simulink model "hopper_6dof_NED_fault_injection"  (R2026a)
settings: Solver=FixedStepAuto  StopTime=30  FixedStep=1e-3  RelTol=1e-5
values from neighbouring files (symbols this model uses):
  cg_init = MP.cg_init    [cg_moi_test.m]
  dcg_dMfu_table = [-0.00217262899893 -0.00217440598527 -0.00217621044518 -0.00217804213665 -0.0021799008032 -0.00218178621725 -0.00218369812677 -0.0021856362975 -0.00218760049076 -0.00218959047338 -0.00219160600889 -0.0021936468686 ... (10000 elements, 100x100)]    [cg_I_LUT.mat]    (also in cg_moi_table_generation.m = MP.dcg_dMfu_table; cg_moi_test.m = MP.dcg_dMfu_table)
  dcg_dMox_table = [0.00344752331682 0.00347104712195 0.00349447366155 0.00351780347518 0.00354103709244 0.00356417504177 0.00358721784832 0.00361016603279 0.00363302011142 0.00365578059713 0.00367844800397 0.0037010228382 ... (10000 elements, 100x100)]    [cg_I_LUT.mat]    (also in cg_moi_table_generation.m = MP.dcg_dMox_table; cg_moi_test.m = MP.dcg_dMox_table)
  dI_dMfu_table = [0.00582660125037 0.00582660125148 0.00582660125148 0.00582660125037 0.00582660125037 0.00582660124926 0.00582660124926 0.00582660125037 0.00582660125037 0.00582660125148 0.00582660125148 0.00582660125037 ... (90000 elements, 100x100x9)]    [cg_I_LUT.mat]    (also in cg_moi_table_generation.m = MP.dI_dMfu_table; cg_moi_test.m = MP.dI_dMfu_table)
  dI_dMox_table = [0.00582660125037 0.00582660124926 0.00582660125037 0.00582660124926 0.00582660125037 0.00582660124926 0.00582660125037 0.00582660124926 0.00582660125037 0.00582660125037 0.00582660125037 0.00582660125037 ... (90000 elements, 100x100x9)]    [cg_I_LUT.mat]    (also in cg_moi_table_generation.m = MP.dI_dMox_table; cg_moi_test.m = MP.dI_dMox_table)
  engine_cg = IN.engine_cg    [cg_moi_test.m]
  engine_mass = IN.engine_mass    [cg_moi_test.m]
  fu_masses = [0 0.131313131313 0.262626262626 0.393939393939 0.525252525253 0.656565656566 0.787878787879 0.919191919192 1.05050505051 1.18181818182 1.31313131313 1.44444444444 ... (100 elements, 1x100)]    [cg_I_LUT.mat]    (also in cg_moi_table_generation.m = MP.fu_masses; cg_moi_test.m = MP.fu_masses)
  g = p.g    [HopperLinearization_6DOF.m]    (also in HopperLinearization_6DOF_LQR.m; HopperLinearization_6DOF_inertial.m; HopperLinearization_errorq.m; TetherTrajectory.m = 9.81)
  K1flat = zeros(N,52)    [GenerateLQ.m]    (also in LQTrack_Master.m = zeros(length(tgrid),48); LinerizationMaster.m = zeros(length(tgrid),52))
  K2grid = GainTable.K2'    [GenerateLQ.m]    (also in LQTrack_Master.m; LinerizationMaster.m)
  MoI_init = MP.MoI_init    [cg_moi_test.m]
  mount_cg = IN.mount_cg    [cg_moi_test.m]
  ox_masses = [0 0.161616161616 0.323232323232 0.484848484848 0.646464646465 0.808080808081 0.969696969697 1.13131313131 1.29292929293 1.45454545455 1.61616161616 1.77777777778 ... (100 elements, 1x100)]    [cg_I_LUT.mat]    (also in cg_moi_table_generation.m = MP.ox_masses; cg_moi_test.m = MP.ox_masses)
  tank_r = 0.10795    [baffle_lut.mat]    (also in cg_moi_test.m = TANKS.singular.radius)
  Target_Trajectory = [0 0 0 0 0 0 0 0 0 sqrt(2)/2 0 sqrt(2)/2 0]'    [LQGeneral.m]    (also in LQTrack_Master.m = [x_trajectory; y_trajectory; z_trajectory;                  ; LinerizationMaster.m = [x_trajectory;y_trajectory;z_trajectory;    vx_trajectory;vy)
  tgrid = t    [LQTrack_Master.m]    (also in LinerizationMaster.m; Trajectory3.m = [t1 t2 t3]'; TrajectoryFollowingGains.m = tgrid(:); TrajectoryFollowingGains2.m = tgrid(:))
  unom = [T_profile, delta_y_profile, delta_z_profile, rcsp]    [LQTrack_Master.m]    (also in LinerizationMaster.m; Trajectory3.m = [; TrajectoryFollowingGains.m = [T_profile(:), zeros(N,1)])
undefined symbols (not defined in the file or in its folder): ENGINE, fu_axial_damping_ratios, fu_lateral_damping_ratios, fu_mass_profile, fu_mdot_data, IN, OUT, ox_axial_damping_ratios, ox_lateral_damping_ratios, ox_mass_profile, ox_mdot_data, pressureLevels, r_leg_1, r_leg_2, r_leg_3, r_leg_4, TANKS, thrust_data, uwndTable, VEH, vwndTable
libraries: fl_lib x31, nesl_utility x25, matrix_library x18, SimscapeFluids_lib x10, simulink_extras x7, slpidlib x7, simulink x7, dspindex x3, aerolibanim x1, commrandsrc3 x1, aerolibutil x1, dspsrcs4 x1
(part 6 of 7)

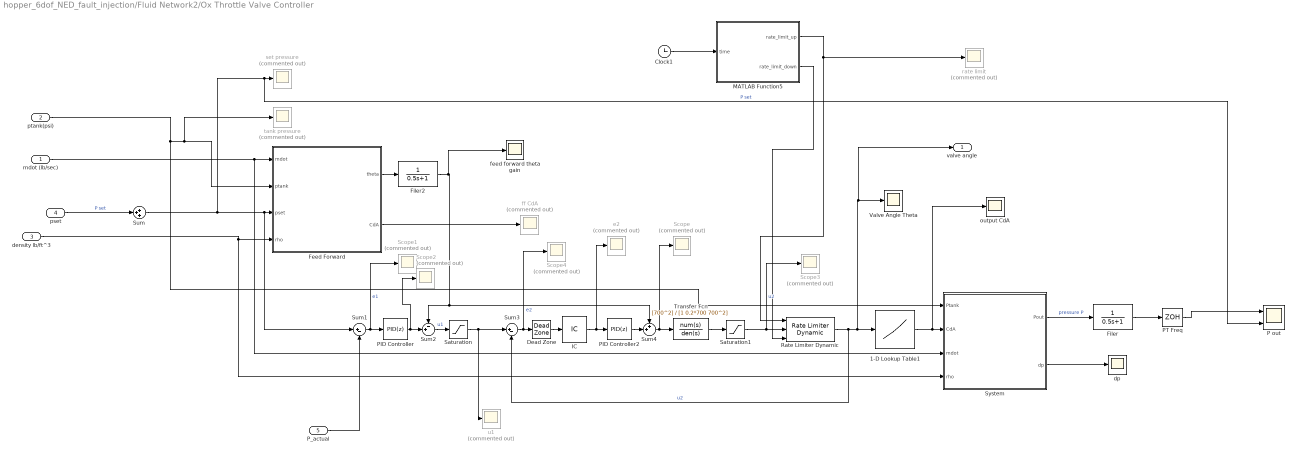
== system hopper_6dof_NED_fault_injection/Fluid Network2/Ox Throttle Valve Controller ==
  mdot (lb/sec) : Inport
  ptank(psi) : Inport  Port=2
  density lb/ft^3 : Inport  Port=3
  pset : Inport  Port=4
  P_actual : Inport  Port=5
  1-D Lookup Table1 : Lookup_n-D  NumberOfTableDimensions=1  BreakpointsForDimension1=[27, 36, 45, 54, 63, 72, 81, 90]  Table="[0.01,  0.06, 0.21, 0.46, 0.83, 1.35, 2.04, 2.93] ./ 37.97"  ExtrapMethod=Clip  InternalRulePriority=Speed  RndMeth=Simplest
  Clock1 : Clock
  Dead Zone : DeadZone  LowerValue=-30  UpperValue=30
  Feed Forward : MATLAB Function  TreatAsAtomicUnit=on
  Filer : TransferFcn  Denominator=[0.5 1]
  Filer2 : TransferFcn  Denominator=[0.5 1]
  IC : InitialCondition  Value=0
  MATLAB Function5 : MATLAB Function  TreatAsAtomicUnit=on
  P out : Scope  NumInputPorts=2
      settings: ActiveDisplayYMinimum=-153.57845403205533  ActiveDisplayYMaximum=515.02423080214487  DataLoggingVariableName=ScopeData20
  PID Controller : slpidlib/PID Controller  Controller=PID  Form=Parallel  TimeDomain=Discrete-time  UseExternalTs=off  SampleTime=0.01  IntegratorMethod=Forward Euler  FilterMethod=Forward Euler  ControllerParametersSource=internal  P=6  I=0.5  UseKiTs=off  D=0  UseExternalDerivativeSource=off  N=100  UseFilter=on  TunerSelectOption=Transfer Function Based (PID Tuner App)  InitialConditionSource=internal  InitialConditionForIntegrator=0  InitialConditionForFilter=0  DifferentiatorICPrevScaledInput=0  ExternalReset=none  TrackingMode=off  Kt=1  LimitOutput=off  SatLimitsSource=internal  UpperSaturationLimit=inf  LowerSaturationLimit=-inf  LinearizeAsGain=on  AntiWindupMode=none  Kb=1  LimitIntegrator=off  UpperIntegratorSaturationLimit=inf  LowerIntegratorSaturationLimit=-inf  POutMin=[]  POutMax=[]  IOutMin=[]  IOutMax=[]  DOutMin=[]  DOutMax=[]  NOutMin=[]  NOutMax=[]  SumOutMin=[]  SumOutMax=[]  SaturationOutMin=[]  SaturationOutMax=[]  PParamMin=[]  PParamMax=[]  IParamMin=[]  IParamMax=[]  DParamMin=[]  DParamMax=[]  NParamMin=[]  NParamMax=[]  KbParamMin=[]  KbParamMax=[]  KtParamMin=[]  KtParamMax=[]  KbOutMin=[]  KbOutMax=[]  KtOutMin=[]  KtOutMax=[]  IntegratorOutMin=[]  IntegratorOutMax=[]  FilterOutMin=[]  FilterOutMax=[]  SumI1OutMin=[]  SumI1OutMax=[]  SumI2OutMin=[]  SumI2OutMax=[]  SumI3OutMin=[]  SumI3OutMax=[]  SumI4OutMin=[]  SumI4OutMax=[]  SumDOutMin=[]  SumDOutMax=[]  DifferentiatorOutMin=[]  DifferentiatorOutMax=[]  FilterDiffOutCoefMin=[]  FilterDiffOutCoefMax=[]  ReciprocalOutMin=[]  ReciprocalOutMax=[]  SumDenOutMin=[]  SumDenOutMax=[]  SumNumOutMin=[]  SumNumOutMax=[]  DivideOutMin=[]  DivideOutMax=[]  UdiffTsProdOutMin=[]  UdiffTsProdOutMax=[]  NTsProdOutMin=[]  NTsProdOutMax=[]  UintegralTsProdOutMin=[]  UintegralTsProdOutMax=[]  UngainTsProdOutMin=[]  UngainTsProdOutMax=[]  ClampingZeroOutDataTypeStr=Inherit: Inherit via back propagation  ClampingZeroOutMin=[]  ClampingZeroOutMax=[]  FilterDenConstantOutDataTypeStr=Inherit: Inherit via back propagation  FilterDenConstantOutMin=[]  FilterDenConstantOutMax=[]  PCopyOutDataTypeStr=Inherit: Inherit via back propagation  PCopyOutMin=[]  PCopyOutMax=[]  NCopyOutDataTypeStr=Inherit: Inherit via back propagation  NCopyOutMin=[]  NCopyOutMax=[]  IntegratorContinuousStateAttributes=''  IntegratorStateMustResolveToSignalObject=off  IntegratorRTWStateStorageClass=Auto  FilterContinuousStateAttributes=''  FilterStateMustResolveToSignalObject=off  FilterRTWStateStorageClass=Auto  ParallelPVariant=InternalParameters  IdealPVariant=Disabled  IVariant=InternalParameters  DVariant=InternalParameters  IntegratorVariant=Discrete  SatVariant=Disabled  AWVariant=Passthrough  PCopyVariant=Disabled  TRVariant=Disabled  FdbkBlocksVariant=Forward  IdealPFdbkVariant=Disabled  SatFdbkVariant=Disabled  DerivativeFilterVariant=ForwardEulerFilter  NVariant=InternalParameters  NCopyVariant=Disabled  FilterICVariant=InternalICsFilter  IntegratorICVariant=InternalICs  ExternalResetVariant=Disabled  TRSumVariant=Passthrough  SumFdbkVariant=Disabled  SumVariant=Sum_PID  TsampFilterVariant=InternalTs  TsampNgainVariant=Passthrough  TsampIntegralVariant=Disabled_SignalSpec  ExternalSaturationOutDataTypeStr=Inherit: Same as second input  DerivativeSourceVariant=ErrorSignal  PreIntVariant=InternalPreInt
  PID Controller2 : slpidlib/PID Controller  Controller=PID  Form=Parallel  TimeDomain=Discrete-time  UseExternalTs=off  SampleTime=0.001  IntegratorMethod=Forward Euler  FilterMethod=Forward Euler  ControllerParametersSource=internal  P=0.1  I=0.6  UseKiTs=off  D=0  UseExternalDerivativeSource=off  N=100  UseFilter=on  TunerSelectOption=Transfer Function Based (PID Tuner App)  InitialConditionSource=internal  InitialConditionForIntegrator=0  InitialConditionForFilter=0  DifferentiatorICPrevScaledInput=0  ExternalReset=none  TrackingMode=off  Kt=1  LimitOutput=off  SatLimitsSource=internal  UpperSaturationLimit=inf  LowerSaturationLimit=-inf  LinearizeAsGain=on  AntiWindupMode=none  Kb=1  LimitIntegrator=off  UpperIntegratorSaturationLimit=inf  LowerIntegratorSaturationLimit=-inf  POutMin=[]  POutMax=[]  IOutMin=[]  IOutMax=[]  DOutMin=[]  DOutMax=[]  NOutMin=[]  NOutMax=[]  SumOutMin=[]  SumOutMax=[]  SaturationOutMin=[]  SaturationOutMax=[]  PParamMin=[]  PParamMax=[]  IParamMin=[]  IParamMax=[]  DParamMin=[]  DParamMax=[]  NParamMin=[]  NParamMax=[]  KbParamMin=[]  KbParamMax=[]  KtParamMin=[]  KtParamMax=[]  KbOutMin=[]  KbOutMax=[]  KtOutMin=[]  KtOutMax=[]  IntegratorOutMin=[]  IntegratorOutMax=[]  FilterOutMin=[]  FilterOutMax=[]  SumI1OutMin=[]  SumI1OutMax=[]  SumI2OutMin=[]  SumI2OutMax=[]  SumI3OutMin=[]  SumI3OutMax=[]  SumI4OutMin=[]  SumI4OutMax=[]  SumDOutMin=[]  SumDOutMax=[]  DifferentiatorOutMin=[]  DifferentiatorOutMax=[]  FilterDiffOutCoefMin=[]  FilterDiffOutCoefMax=[]  ReciprocalOutMin=[]  ReciprocalOutMax=[]  SumDenOutMin=[]  SumDenOutMax=[]  SumNumOutMin=[]  SumNumOutMax=[]  DivideOutMin=[]  DivideOutMax=[]  UdiffTsProdOutMin=[]  UdiffTsProdOutMax=[]  NTsProdOutMin=[]  NTsProdOutMax=[]  UintegralTsProdOutMin=[]  UintegralTsProdOutMax=[]  UngainTsProdOutMin=[]  UngainTsProdOutMax=[]  ClampingZeroOutDataTypeStr=Inherit: Inherit via back propagation  ClampingZeroOutMin=[]  ClampingZeroOutMax=[]  FilterDenConstantOutDataTypeStr=Inherit: Inherit via back propagation  FilterDenConstantOutMin=[]  FilterDenConstantOutMax=[]  PCopyOutDataTypeStr=Inherit: Inherit via back propagation  PCopyOutMin=[]  PCopyOutMax=[]  NCopyOutDataTypeStr=Inherit: Inherit via back propagation  NCopyOutMin=[]  NCopyOutMax=[]  IntegratorContinuousStateAttributes=''  IntegratorStateMustResolveToSignalObject=off  IntegratorRTWStateStorageClass=Auto  FilterContinuousStateAttributes=''  FilterStateMustResolveToSignalObject=off  FilterRTWStateStorageClass=Auto  ParallelPVariant=InternalParameters  IdealPVariant=Disabled  IVariant=InternalParameters  DVariant=InternalParameters  IntegratorVariant=Discrete  SatVariant=Disabled  AWVariant=Passthrough  PCopyVariant=Disabled  TRVariant=Disabled  FdbkBlocksVariant=Forward  IdealPFdbkVariant=Disabled  SatFdbkVariant=Disabled  DerivativeFilterVariant=ForwardEulerFilter  NVariant=InternalParameters  NCopyVariant=Disabled  FilterICVariant=InternalICsFilter  IntegratorICVariant=InternalICs  ExternalResetVariant=Disabled  TRSumVariant=Passthrough  SumFdbkVariant=Disabled  SumVariant=Sum_PID  TsampFilterVariant=InternalTs  TsampNgainVariant=Passthrough  TsampIntegralVariant=Disabled_SignalSpec  ExternalSaturationOutDataTypeStr=Inherit: Same as second input  DerivativeSourceVariant=ErrorSignal  PreIntVariant=InternalPreInt
  PT Freq : ZeroOrderHold  SampleTime=1/200
  Rate Limiter Dynamic : simulink/Discontinuities/Rate Limiter Dynamic
  Saturation : Saturate  UpperLimit=90  LowerLimit=0
  Saturation1 : Saturate  UpperLimit=90  LowerLimit=0
  Scope{,1..4} (5 alike) : Scope  Commented=on
      Scope settings: ActiveDisplayYMinimum=-275.11641924282065  ActiveDisplayYMaximum=563.35245614782866  DataLoggingVariableName=ScopeData23
      Scope1 settings: ActiveDisplayYMinimum=-63.640747784829  ActiveDisplayYMaximum=395.9600830872032  DataLoggingVariableName=ScopeData24
      Scope2 settings: ActiveDisplayYMinimum=-1  ActiveDisplayYMaximum=1  DataLoggingVariableName=ScopeData25
      Scope3 settings: ActiveDisplayYMinimum=-1  ActiveDisplayYMaximum=1  DataLoggingVariableName=ScopeData26
      Scope4 settings: ActiveDisplayYMinimum=-1  ActiveDisplayYMaximum=1  DataLoggingVariableName=ScopeData27
  Sum : Sum  Inputs=+++
  Sum1 : Sum  Inputs=|+-
  Sum2 : Sum  Inputs=-+|
  Sum3 : Sum  Inputs=|+-
  Sum4 : Sum  Inputs=++|
  System : MATLAB Function  TreatAsAtomicUnit=on
  Transfer Fcn : TransferFcn  Numerator=[700^2]  Denominator=[1 0.2*700 700^2]
  Valve Angle Theta : Scope
      settings: ActiveDisplayYMinimum=-54.50975234839  ActiveDisplayYMaximum=77.0496336171224
  dp : Scope
      settings: ActiveDisplayYMinimum=-18119.240749435841  ActiveDisplayYMaximum=163753.70976632342  DataLoggingVariableName=ScopeData28
  e2 : Scope  Commented=on
      settings: ActiveDisplayYMinimum=-94.713391249832966  ActiveDisplayYMaximum=253.61308310962266  DataLoggingVariableName=ScopeData29
  feed forward theta gain : Scope
      settings: ActiveDisplayYMinimum=36.144112332478429  ActiveDisplayYMaximum=40.8018145520034  DataLoggingVariableName=ScopeData2
  ff CdA : Scope  Commented=on
      settings: ActiveDisplayYMinimum=0.00619  ActiveDisplayYMaximum=0.00757  DataLoggingVariableName=ScopeData30
  output CdA : Scope
      settings: ActiveDisplayYMinimum=-0.0014226243070618195  ActiveDisplayYMaximum=0.015437276914728357  DataLoggingVariableName=ScopeData3
  rate limit : Scope  Commented=on
      settings: ActiveDisplayYMinimum=-1  ActiveDisplayYMaximum=1  DataLoggingVariableName=ScopeData31
  set pressure : Scope  Commented=on
      settings: ActiveDisplayYMinimum=-1  ActiveDisplayYMaximum=1  DataLoggingVariableName=ScopeData32
  tank pressure : Scope  Commented=on
      settings: ActiveDisplayYMinimum=243.75  ActiveDisplayYMaximum=306.25  DataLoggingVariableName=ScopeData33
  u1 : Scope  Commented=on
      settings: ActiveDisplayYMinimum=-1  ActiveDisplayYMaximum=1  DataLoggingVariableName=ScopeData34
  valve angle : Outport
  wires:
  Sum3/1 -> Dead Zone/1, Scope4/1  "e2"
  density lb/ft^3/1 -> System/4(rho), Feed Forward/4(rho)
  Filer/1 -> PT Freq/1
  Sum/1 -> P out/2, set pressure/1, Sum1/1, Feed Forward/3(pset)  "P set"
  ptank(psi)/1 -> System/1(Ptank), Feed Forward/2(ptank), tank pressure/1
  PID Controller/1 -> Scope2/1, Sum2/2
  PT Freq/1 -> P out/1
  Transfer Fcn/1 -> Saturation1/1
  IC/1 -> PID Controller2/1, e2/1
  Feed Forward/1(theta) -> Filer2/1
  MATLAB Function5/2(rate_limit_down) -> Rate Limiter Dynamic/3
  Dead Zone/1 -> IC/1
  Rate Limiter Dynamic/1 -> valve angle/1, Valve Angle Theta/1, 1-D Lookup Table1/1, Sum3/2  "u2"
  pset/1 -> Sum/2  "P set"
  Sum4/1 -> Scope/1, Transfer Fcn/1
  Saturation1/1 -> Scope3/1, Rate Limiter Dynamic/2  "u2"
  mdot (lb/sec)/1 -> System/3(mdot), Feed Forward/1(mdot)
  MATLAB Function5/1(rate_limit_up) -> Rate Limiter Dynamic/1, rate limit/1
  Clock1/1 -> MATLAB Function5/1(time)
  1-D Lookup Table1/1 -> System/2(CdA), output CdA/1
  PID Controller2/1 -> Sum4/2
  Sum1/1 -> Scope1/1, PID Controller/1  "e1"
  Sum2/1 -> Saturation/1  "u1"
  Feed Forward/2(CdA) -> ff CdA/1
  System/2(dp) -> dp/1
  Saturation/1 -> u1/1, Sum3/1
  System/1(Pout) -> Filer/1  "pressure P"
  Filer2/1 -> Sum4/1, Sum2/1, feed forward theta gain/1
  P_actual/1 -> Sum1/2

== system hopper_6dof_NED_fault_injection/Fluid Network2/Physical Combustion Chamber ==
  pc : Inport
  Local Restriction (TL) : fl_lib/Thermal Liquid/Elements/Local Restriction (TL)  Commented=through  restriction_type=foundation.enum.restriction_type.fixed  restriction_area=0.001 m^2  min_area=1e-10 m^2  max_area=0.005 m^2  area=0.01 m^2  Cd=0.64  Re_c=150  pressure_recovery=true
  Local Restriction (TL)1 : fl_lib/Thermal Liquid/Elements/Local Restriction (TL)  Commented=through  restriction_type=foundation.enum.restriction_type.fixed  restriction_area=0.001 m^2  min_area=1e-10 m^2  max_area=0.005 m^2  area=0.01 m^2  Cd=0.64  Re_c=150  pressure_recovery=true
  Pressure Source (TL) : fl_lib/Thermal Liquid/Sources/Pressure Source (TL)  source_type=foundation.enum.constant_controlled.controlled  pressure_differential=0 MPa  power_spec=foundation.enum.power_spec.isentropic  area=0.01 m^2
      settings: InternalSimscapePortConfiguration="{\"Bottom\":[],\"Left\":[{\"id\":\"A\",\"label\":\"A\",\"type\":\"foundation.thermal_liquid.thermal_liquid\"},{\"id\":\"P\",\"label\":\"P\",\"type\":\"input\"}],\"Right\":[{\"id\":\"B\",\"label\":\"B\",\"type\":\"foundation.thermal_liquid.thermal_liquid\"}],\"Top\":[]}"
  Pressure Source (TL)1 : fl_lib/Thermal Liquid/Sources/Pressure Source (TL)  source_type=foundation.enum.constant_controlled.controlled  pressure_differential=0 MPa  power_spec=foundation.enum.power_spec.isentropic  area=0.01 m^2
      settings: InternalSimscapePortConfiguration="{\"Bottom\":[],\"Left\":[{\"id\":\"A\",\"label\":\"A\",\"type\":\"foundation.thermal_liquid.thermal_liquid\"},{\"id\":\"P\",\"label\":\"P\",\"type\":\"input\"}],\"Right\":[{\"id\":\"B\",\"label\":\"B\",\"type\":\"foundation.thermal_liquid.thermal_liquid\"}],\"Top\":[]}"
  Reservoir (TL) : fl_lib/Thermal Liquid/Elements/Reservoir (TL)  pressure_spec=foundation.enum.pressure_spec.atmospheric  reservoir_pressure=0.101325 MPa  reservoir_temperature=293.15 K  area=0.01 m^2
  Reservoir (TL)1 : fl_lib/Thermal Liquid/Elements/Reservoir (TL)  pressure_spec=foundation.enum.pressure_spec.atmospheric  reservoir_pressure=0.101325 MPa  reservoir_temperature=100 K  area=0.01 m^2
  Simulink-PS Converter1 : nesl_utility/Simulink-PS Converter  PhysicalDomain=network_engine_domain  SubClassName=ps_input  LeftPortType=input  RightPortType=output  PseudoPeriodic=off  Frequencies=[]  NoiseDistribution=none  NoiseParameters=[]  Unit=1  AffineConversion=off  FilteringAndDerivatives=filter  SimscapeFilterOrder=1  InputFilterTimeConstant=0.001  UdotUserProvided=0
  Simulink-PS Converter4 : nesl_utility/Simulink-PS Converter  PhysicalDomain=network_engine_domain  SubClassName=ps_input  LeftPortType=input  RightPortType=output  PseudoPeriodic=off  Frequencies=[]  NoiseDistribution=none  NoiseParameters=[]  Unit=1  AffineConversion=off  FilteringAndDerivatives=filter  SimscapeFilterOrder=1  InputFilterTimeConstant=0.001  UdotUserProvided=0
  fuel line : PMIOPort  Side=Right
  ox line : PMIOPort  Port=2  Side=Right
  wires:
  pc/1 -> Simulink-PS Converter1/1, Simulink-PS Converter4/1
  connections:
  Simulink-PS Converter4/RConn1 -- Pressure Source (TL)/LConn2
  Simulink-PS Converter1/RConn1 -- Pressure Source (TL)1/LConn2
  Local Restriction (TL)/LConn1 -- Pressure Source (TL)/LConn1
  Reservoir (TL)/LConn1 -- Local Restriction (TL)/RConn1
  fuel line/RConn1 -- Pressure Source (TL)/RConn1
  Local Restriction (TL)1/LConn1 -- Pressure Source (TL)1/LConn1
  Reservoir (TL)1/LConn1 -- Local Restriction (TL)1/RConn1
  Pressure Source (TL)1/RConn1 -- ox line/RConn1

== system hopper_6dof_NED_fault_injection/Fluid Network2/fuel mdot feedback//corrections ==
  actual mdot : Inport
  commanded mdot : Inport  Port=2
  MR correction : Inport  Port=3
  PID Controller1 : slpidlib/PID Controller  Controller=PID  Form=Parallel  TimeDomain=Continuous-time  UseExternalTs=off  SampleTime=-1  IntegratorMethod=Forward Euler  FilterMethod=Forward Euler  ControllerParametersSource=internal  P=1  I=1  UseKiTs=off  D=0  UseExternalDerivativeSource=off  N=20  UseFilter=on  TunerSelectOption=Transfer Function Based (PID Tuner App)  InitialConditionSource=internal  InitialConditionForIntegrator=0  InitialConditionForFilter=0  DifferentiatorICPrevScaledInput=0  ExternalReset=none  TrackingMode=off  Kt=1  LimitOutput=off  SatLimitsSource=internal  UpperSaturationLimit=inf  LowerSaturationLimit=-inf  LinearizeAsGain=on  AntiWindupMode=none  Kb=1  LimitIntegrator=off  UpperIntegratorSaturationLimit=inf  LowerIntegratorSaturationLimit=-inf  POutMin=[]  POutMax=[]  IOutMin=[]  IOutMax=[]  DOutMin=[]  DOutMax=[]  NOutMin=[]  NOutMax=[]  SumOutMin=[]  SumOutMax=[]  SaturationOutMin=[]  SaturationOutMax=[]  PParamMin=[]  PParamMax=[]  IParamMin=[]  IParamMax=[]  DParamMin=[]  DParamMax=[]  NParamMin=[]  NParamMax=[]  KbParamMin=[]  KbParamMax=[]  KtParamMin=[]  KtParamMax=[]  KbOutMin=[]  KbOutMax=[]  KtOutMin=[]  KtOutMax=[]  IntegratorOutMin=[]  IntegratorOutMax=[]  FilterOutMin=[]  FilterOutMax=[]  SumI1OutMin=[]  SumI1OutMax=[]  SumI2OutMin=[]  SumI2OutMax=[]  SumI3OutMin=[]  SumI3OutMax=[]  SumI4OutMin=[]  SumI4OutMax=[]  SumDOutMin=[]  SumDOutMax=[]  DifferentiatorOutMin=[]  DifferentiatorOutMax=[]  FilterDiffOutCoefMin=[]  FilterDiffOutCoefMax=[]  ReciprocalOutMin=[]  ReciprocalOutMax=[]  SumDenOutMin=[]  SumDenOutMax=[]  SumNumOutMin=[]  SumNumOutMax=[]  DivideOutMin=[]  DivideOutMax=[]  UdiffTsProdOutMin=[]  UdiffTsProdOutMax=[]  NTsProdOutMin=[]  NTsProdOutMax=[]  UintegralTsProdOutMin=[]  UintegralTsProdOutMax=[]  UngainTsProdOutMin=[]  UngainTsProdOutMax=[]  ClampingZeroOutDataTypeStr=Inherit: Inherit via back propagation  ClampingZeroOutMin=[]  ClampingZeroOutMax=[]  FilterDenConstantOutDataTypeStr=Inherit: Inherit via back propagation  FilterDenConstantOutMin=[]  FilterDenConstantOutMax=[]  PCopyOutDataTypeStr=Inherit: Inherit via back propagation  PCopyOutMin=[]  PCopyOutMax=[]  NCopyOutDataTypeStr=Inherit: Inherit via back propagation  NCopyOutMin=[]  NCopyOutMax=[]  IntegratorContinuousStateAttributes=''  IntegratorStateMustResolveToSignalObject=off  IntegratorRTWStateStorageClass=Auto  FilterContinuousStateAttributes=''  FilterStateMustResolveToSignalObject=off  FilterRTWStateStorageClass=Auto  ParallelPVariant=InternalParameters  IdealPVariant=Disabled  IVariant=InternalParameters  DVariant=InternalParameters  IntegratorVariant=Continuous  SatVariant=Disabled  AWVariant=Passthrough  PCopyVariant=Disabled  TRVariant=Disabled  FdbkBlocksVariant=Forward  IdealPFdbkVariant=Disabled  SatFdbkVariant=Disabled  DerivativeFilterVariant=ContFilter  NVariant=InternalParameters  NCopyVariant=Disabled  FilterICVariant=InternalICsFilter  IntegratorICVariant=InternalICs  ExternalResetVariant=Disabled  TRSumVariant=Passthrough  SumFdbkVariant=Disabled  SumVariant=Sum_PID  TsampFilterVariant=InternalTs  TsampNgainVariant=Passthrough  TsampIntegralVariant=Disabled_SignalSpec  ExternalSaturationOutDataTypeStr=Inherit: Same as second input  DerivativeSourceVariant=ErrorSignal  PreIntVariant=InternalPreInt
  Sum2 : Sum  Inputs=|+-
  Sum3 : Sum  Inputs=|+-
  Sum4 : Sum  Inputs=|++
  kg/s to lb/s1 : Gain  Gain=2.20462
  fuel mdot : Outport
  wires:
  MR correction/1 -> Sum2/2
  Sum2/1 -> Sum4/2, Sum3/1
  PID Controller1/1 -> Sum4/1
  Sum3/1 -> PID Controller1/1
  Sum4/1 -> kg/s to lb/s1/1
  commanded mdot/1 -> Sum2/1
  actual mdot/1 -> Sum3/2
  kg/s to lb/s1/1 -> fuel mdot/1

== system hopper_6dof_NED_fault_injection/Fluid Network2/ox mdot feedback//corrections ==
  commanded mdot : Inport
  actual mdot : Inport  Port=2
  PID Controller2 : slpidlib/PID Controller  Controller=PID  Form=Parallel  TimeDomain=Continuous-time  UseExternalTs=off  SampleTime=-1  IntegratorMethod=Forward Euler  FilterMethod=Forward Euler  ControllerParametersSource=internal  P=1  I=1  UseKiTs=off  D=0  UseExternalDerivativeSource=off  N=20  UseFilter=on  TunerSelectOption=Transfer Function Based (PID Tuner App)  InitialConditionSource=internal  InitialConditionForIntegrator=0  InitialConditionForFilter=0  DifferentiatorICPrevScaledInput=0  ExternalReset=none  TrackingMode=off  Kt=1  LimitOutput=off  SatLimitsSource=internal  UpperSaturationLimit=inf  LowerSaturationLimit=-inf  LinearizeAsGain=on  AntiWindupMode=none  Kb=1  LimitIntegrator=off  UpperIntegratorSaturationLimit=inf  LowerIntegratorSaturationLimit=-inf  POutMin=[]  POutMax=[]  IOutMin=[]  IOutMax=[]  DOutMin=[]  DOutMax=[]  NOutMin=[]  NOutMax=[]  SumOutMin=[]  SumOutMax=[]  SaturationOutMin=[]  SaturationOutMax=[]  PParamMin=[]  PParamMax=[]  IParamMin=[]  IParamMax=[]  DParamMin=[]  DParamMax=[]  NParamMin=[]  NParamMax=[]  KbParamMin=[]  KbParamMax=[]  KtParamMin=[]  KtParamMax=[]  KbOutMin=[]  KbOutMax=[]  KtOutMin=[]  KtOutMax=[]  IntegratorOutMin=[]  IntegratorOutMax=[]  FilterOutMin=[]  FilterOutMax=[]  SumI1OutMin=[]  SumI1OutMax=[]  SumI2OutMin=[]  SumI2OutMax=[]  SumI3OutMin=[]  SumI3OutMax=[]  SumI4OutMin=[]  SumI4OutMax=[]  SumDOutMin=[]  SumDOutMax=[]  DifferentiatorOutMin=[]  DifferentiatorOutMax=[]  FilterDiffOutCoefMin=[]  FilterDiffOutCoefMax=[]  ReciprocalOutMin=[]  ReciprocalOutMax=[]  SumDenOutMin=[]  SumDenOutMax=[]  SumNumOutMin=[]  SumNumOutMax=[]  DivideOutMin=[]  DivideOutMax=[]  UdiffTsProdOutMin=[]  UdiffTsProdOutMax=[]  NTsProdOutMin=[]  NTsProdOutMax=[]  UintegralTsProdOutMin=[]  UintegralTsProdOutMax=[]  UngainTsProdOutMin=[]  UngainTsProdOutMax=[]  ClampingZeroOutDataTypeStr=Inherit: Inherit via back propagation  ClampingZeroOutMin=[]  ClampingZeroOutMax=[]  FilterDenConstantOutDataTypeStr=Inherit: Inherit via back propagation  FilterDenConstantOutMin=[]  FilterDenConstantOutMax=[]  PCopyOutDataTypeStr=Inherit: Inherit via back propagation  PCopyOutMin=[]  PCopyOutMax=[]  NCopyOutDataTypeStr=Inherit: Inherit via back propagation  NCopyOutMin=[]  NCopyOutMax=[]  IntegratorContinuousStateAttributes=''  IntegratorStateMustResolveToSignalObject=off  IntegratorRTWStateStorageClass=Auto  FilterContinuousStateAttributes=''  FilterStateMustResolveToSignalObject=off  FilterRTWStateStorageClass=Auto  ParallelPVariant=InternalParameters  IdealPVariant=Disabled  IVariant=InternalParameters  DVariant=InternalParameters  IntegratorVariant=Continuous  SatVariant=Disabled  AWVariant=Passthrough  PCopyVariant=Disabled  TRVariant=Disabled  FdbkBlocksVariant=Forward  IdealPFdbkVariant=Disabled  SatFdbkVariant=Disabled  DerivativeFilterVariant=ContFilter  NVariant=InternalParameters  NCopyVariant=Disabled  FilterICVariant=InternalICsFilter  IntegratorICVariant=InternalICs  ExternalResetVariant=Disabled  TRSumVariant=Passthrough  SumFdbkVariant=Disabled  SumVariant=Sum_PID  TsampFilterVariant=InternalTs  TsampNgainVariant=Passthrough  TsampIntegralVariant=Disabled_SignalSpec  ExternalSaturationOutDataTypeStr=Inherit: Same as second input  DerivativeSourceVariant=ErrorSignal  PreIntVariant=InternalPreInt
  Sum1 : Sum  Inputs=|+-
  Sum5 : Sum  Inputs=|++
  kg/s to lb/s : Gain  Gain=2.20462
  ox mdot : Outport
  wires:
  Sum1/1 -> PID Controller2/1
  commanded mdot/1 -> Sum5/2, Sum1/1
  PID Controller2/1 -> Sum5/1
  Sum5/1 -> kg/s to lb/s/1
  kg/s to lb/s/1 -> ox mdot/1
  actual mdot/1 -> Sum1/2

== system hopper_6dof_NED_fault_injection/Ground /Leg 1 Force ==
  Leg Position : Inport
  Leg Velocity : Inport  Port=2
  Demux : Demux  Outputs=3
  Demux1 : Demux  Outputs=3
  If : If  NumInputs=2  IfExpression=u1 > -0.001
  If Action Subsystem : Subsystem  TreatAsAtomicUnit=on
  If Action Subsystem1 : Subsystem  TreatAsAtomicUnit=on
  Merge : Merge
  Leg 1 Force : Outport
  wires:
  Leg Position/1 -> If Action Subsystem/1(Leg Position), Demux/1
  If/2 -> If Action Subsystem1/Action
  If Action Subsystem/1(Leg Force) -> Merge/1
  If Action Subsystem1/1(Out1) -> Merge/2
  Merge/1 -> Leg 1 Force/1
  Leg Velocity/1 -> Demux1/1, If Action Subsystem/2(Leg Velocity)
  If/1 -> If Action Subsystem/Action
  Demux/3 -> If/1
  Demux1/3 -> If/2

== system hopper_6dof_NED_fault_injection/Ground /Leg 1 Force1 ==
  Leg Position : Inport
  Leg Velocity : Inport  Port=2
  Demux : Demux  Outputs=3
  Demux1 : Demux  Outputs=3
  If : If  NumInputs=2  IfExpression=u1 > -0.001
  If Action Subsystem : Subsystem  TreatAsAtomicUnit=on
  If Action Subsystem1 : Subsystem  TreatAsAtomicUnit=on
  Merge : Merge
  Leg 1 Force : Outport
  wires:
  Leg Position/1 -> If Action Subsystem/1(Leg Position), Demux/1
  If/2 -> If Action Subsystem1/Action
  If Action Subsystem/1(Leg Force) -> Merge/1
  If Action Subsystem1/1(Out1) -> Merge/2
  Merge/1 -> Leg 1 Force/1
  Leg Velocity/1 -> Demux1/1, If Action Subsystem/2(Leg Velocity)
  If/1 -> If Action Subsystem/Action
  Demux/3 -> If/1
  Demux1/3 -> If/2

== system hopper_6dof_NED_fault_injection/Ground /Leg 1 Force2 ==
  Leg Position : Inport
  Leg Velocity : Inport  Port=2
  Demux : Demux  Outputs=3
  Demux1 : Demux  Outputs=3
  If : If  NumInputs=2  IfExpression=u1 > -0.001
  If Action Subsystem : Subsystem  TreatAsAtomicUnit=on
  If Action Subsystem1 : Subsystem  TreatAsAtomicUnit=on
  Merge : Merge
  Leg 1 Force : Outport
  wires:
  Leg Position/1 -> If Action Subsystem/1(Leg Position), Demux/1
  If/2 -> If Action Subsystem1/Action
  If Action Subsystem/1(Leg Force) -> Merge/1
  If Action Subsystem1/1(Out1) -> Merge/2
  Merge/1 -> Leg 1 Force/1
  Leg Velocity/1 -> Demux1/1, If Action Subsystem/2(Leg Velocity)
  If/1 -> If Action Subsystem/Action
  Demux/3 -> If/1
  Demux1/3 -> If/2

== system hopper_6dof_NED_fault_injection/Ground /Leg 1 Force3 ==
  Leg Position : Inport
  Leg Velocity : Inport  Port=2
  Demux : Demux  Outputs=3
  Demux1 : Demux  Outputs=3
  If : If  NumInputs=2  IfExpression=u1 > -0.001
  If Action Subsystem : Subsystem  TreatAsAtomicUnit=on
  If Action Subsystem1 : Subsystem  TreatAsAtomicUnit=on
  Merge : Merge
  Leg 1 Force : Outport
  wires:
  Leg Position/1 -> If Action Subsystem/1(Leg Position), Demux/1
  If/2 -> If Action Subsystem1/Action
  If Action Subsystem/1(Leg Force) -> Merge/1
  If Action Subsystem1/1(Out1) -> Merge/2
  Merge/1 -> Leg 1 Force/1
  Leg Velocity/1 -> Demux1/1, If Action Subsystem/2(Leg Velocity)
  If/1 -> If Action Subsystem/Action
  Demux/3 -> If/1
  Demux1/3 -> If/2

== system hopper_6dof_NED_fault_injection/Slosh/Fuel Axial Force ==
  fu_axial_accel : Inport
  fu_axial_damping : Inport  Port=2
  fu_axial_pendulum_l : Inport  Port=3
  fu_axial_natural_freq : Inport  Port=4
  fu_axial_slosh_mass : Inport  Port=5
  x_omega_dot : Inport  Port=6
  IC : InitialCondition  Value=0
  Integrator : Integrator
  Integrator1 : Integrator
  MATLAB Function : MATLAB Function  TreatAsAtomicUnit=on
  MATLAB Function1 : MATLAB Function  TreatAsAtomicUnit=on
  MATLAB Function2 : MATLAB Function  TreatAsAtomicUnit=on
  MATLAB Function3 : MATLAB Function  TreatAsAtomicUnit=on
  MATLAB Function4 : MATLAB Function  TreatAsAtomicUnit=on
  Product : Product
  Sum : Sum  Inputs=|++
  Sum1 : Sum  Inputs=|++
  fu_axial_f : Outport
  fu_slosh_x : Outport  Port=2
  fu_slosh_mass_x : Outport  Port=3
  fu_slosh_torque_x : Outport  Port=4
  wires:
  fu_axial_accel/1 -> MATLAB Function/1(fu_axial_accel)
  fu_axial_pendulum_l/1 -> Product/2, MATLAB Function/2(fu_axial_pendulum_l), MATLAB Function3/3(fu_axial_pendulum_l), MATLAB Function4/3(fu_axial_pendulum_l)
  Integrator/1 -> MATLAB Function2/1(fu_axial_phi_dot), Integrator1/1
  MATLAB Function2/1(velo_term) -> Sum/2
  fu_axial_natural_freq/1 -> MATLAB Function2/2(fu_axial_natural_freq), MATLAB Function1/2(fu_axial_natural_freq)
  fu_axial_damping/1 -> MATLAB Function2/3(fu_axial_damping)
  Integrator1/1 -> IC/1
  Sum/1 -> Sum1/1
  MATLAB Function1/1(ang_term) -> Sum1/2
  MATLAB Function/1(accel_term) -> Sum/1
  Sum1/1 -> Integrator/1, MATLAB Function4/4(slosh_angular_accel), MATLAB Function3/1(fu_axial_phi_ddot)
  fu_axial_slosh_mass/1 -> fu_slosh_mass_x/1, MATLAB Function4/2(fu_axial_slosh_mass), MATLAB Function3/2(fu_axial_slosh_mass)
  MATLAB Function3/1(fu_axial_f) -> fu_axial_f/1
  IC/1 -> Product/1, MATLAB Function1/1(fu_axial_phi)
  Product/1 -> fu_slosh_x/1
  MATLAB Function4/1(x_slosh_torque) -> fu_slosh_torque_x/1
  x_omega_dot/1 -> MATLAB Function4/1(x_omega_dot)

== system hopper_6dof_NED_fault_injection/Slosh/Fuel Pitch Force ==
  fu_yaw_accel : Inport
  fu_lateral_damping : Inport  Port=2
  fu_lateral_pendulum_l : Inport  Port=3
  fu_lateral_natural_freq : Inport  Port=4
  fu_lateral_slosh_mass : Inport  Port=5
  z_omega_dot : Inport  Port=6
  IC : InitialCondition  Value=0
  Integrator : Integrator
  Integrator1 : Integrator
  MATLAB Function : MATLAB Function  TreatAsAtomicUnit=on
  MATLAB Function1 : MATLAB Function  TreatAsAtomicUnit=on
  MATLAB Function2 : MATLAB Function  TreatAsAtomicUnit=on
  MATLAB Function3 : MATLAB Function  TreatAsAtomicUnit=on
  MATLAB Function4 : MATLAB Function  TreatAsAtomicUnit=on
  Product : Product
  Sum : Sum  Inputs=|++
  Sum1 : Sum  Inputs=|++
  fu_yaw_f : Outport
  fu_slosh_z : Outport  Port=2
  fu_slosh_mass_z : Outport  Port=3
  fu_slosh_torque_z : Outport  Port=4
  wires:
  fu_yaw_accel/1 -> MATLAB Function/1(fu_yaw_accel)
  fu_lateral_pendulum_l/1 -> MATLAB Function/2(fu_lateral_pendulum_l), Product/2, MATLAB Function4/3(fu_lateral_pendulum_l), MATLAB Function3/3(fu_lateral_pendulum_l)
  Integrator/1 -> MATLAB Function2/1(fu_yaw_phi_dot), Integrator1/1
  MATLAB Function2/1(velo_term) -> Sum/2
  fu_lateral_natural_freq/1 -> MATLAB Function2/2(fu_lateral_natural_freq), MATLAB Function1/2(fu_lateral_natural_freq)
  fu_lateral_damping/1 -> MATLAB Function2/3(fu_lateral_damping)
  Integrator1/1 -> IC/1
  Sum/1 -> Sum1/1
  MATLAB Function1/1(ang_term) -> Sum1/2
  MATLAB Function/1(accel_term) -> Sum/1
  Sum1/1 -> MATLAB Function4/4(slosh_angular_accel), MATLAB Function3/1(fu_yaw_phi_ddot), Integrator/1
  fu_lateral_slosh_mass/1 -> fu_slosh_mass_z/1, MATLAB Function4/2(fu_lateral_slosh_mass), MATLAB Function3/2(fu_lateral_slosh_mass)
  MATLAB Function3/1(fu_yaw_f) -> fu_yaw_f/1
  IC/1 -> Product/1, MATLAB Function1/1(fu_yaw_phi)
  Product/1 -> fu_slosh_z/1
  MATLAB Function4/1(z_slosh_torque) -> fu_slosh_torque_z/1
  z_omega_dot/1 -> MATLAB Function4/1(z_omega_dot)

== system hopper_6dof_NED_fault_injection/Slosh/Fuel Yaw Force ==
  fu_pitch_accel : Inport
  fu_lateral_damping : Inport  Port=2
  fu_lateral_pendulum_l : Inport  Port=3
  fu_lateral_natural_freq : Inport  Port=4
  fu_lateral_slosh_mass : Inport  Port=5
  y_omega_dot : Inport  Port=6
  IC : InitialCondition  Value=0
  Integrator : Integrator
  Integrator1 : Integrator
  MATLAB Function : MATLAB Function  TreatAsAtomicUnit=on
  MATLAB Function1 : MATLAB Function  TreatAsAtomicUnit=on
  MATLAB Function2 : MATLAB Function  TreatAsAtomicUnit=on
  MATLAB Function3 : MATLAB Function  TreatAsAtomicUnit=on
  MATLAB Function4 : MATLAB Function  TreatAsAtomicUnit=on
  Product : Product
  Sum : Sum  Inputs=|++
  Sum1 : Sum  Inputs=|++
  fu_pitch_f : Outport
  fu_slosh_y : Outport  Port=2
  fu_slosh_mass_y : Outport  Port=3
  fu_slosh_torque_y : Outport  Port=4
  wires:
  fu_pitch_accel/1 -> MATLAB Function/1(fu_pitch_accel)
  fu_lateral_pendulum_l/1 -> MATLAB Function/2(fu_lateral_pendulum_l), Product/2, MATLAB Function4/3(fu_lateral_pendulum_l), MATLAB Function3/3(fu_lateral_pendulum_l)
  Integrator/1 -> MATLAB Function2/1(fu_pitch_phi_dot), Integrator1/1
  MATLAB Function2/1(velo_term) -> Sum/2
  fu_lateral_natural_freq/1 -> MATLAB Function1/2(fu_lateral_natural_freq), MATLAB Function2/2(fu_lateral_natural_freq)
  fu_lateral_damping/1 -> MATLAB Function2/3(fu_lateral_damping)
  Integrator1/1 -> IC/1
  Sum/1 -> Sum1/1
  MATLAB Function1/1(ang_term) -> Sum1/2
  MATLAB Function/1(accel_term) -> Sum/1
  Sum1/1 -> Integrator/1, MATLAB Function4/4(slosh_angular_accel), MATLAB Function3/1(fu_pitch_phi_ddot)
  fu_lateral_slosh_mass/1 -> fu_slosh_mass_y/1, MATLAB Function4/2(fu_lateral_slosh_mass), MATLAB Function3/2(fu_lateral_slosh_mass)
  MATLAB Function3/1(fu_pitch_f) -> fu_pitch_f/1
  IC/1 -> Product/1, MATLAB Function1/1(fu_pitch_phi)
  Product/1 -> fu_slosh_y/1
  y_omega_dot/1 -> MATLAB Function4/1(y_omega_dot)
  MATLAB Function4/1(y_slosh_torque) -> fu_slosh_torque_y/1

== system hopper_6dof_NED_fault_injection/Slosh/Oxidizer Axial Force ==
  ox_axial_accel : Inport
  ox_axial_damping : Inport  Port=2
  ox_axial_pendulum_l : Inport  Port=3
  ox_axial_natural_freq : Inport  Port=4
  ox_axial_slosh_mass : Inport  Port=5
  x_omega_dot : Inport  Port=6
  IC : InitialCondition  Value=0
  Integrator : Integrator
  Integrator1 : Integrator
  MATLAB Function : MATLAB Function  TreatAsAtomicUnit=on
  MATLAB Function1 : MATLAB Function  TreatAsAtomicUnit=on
  MATLAB Function2 : MATLAB Function  TreatAsAtomicUnit=on
  MATLAB Function3 : MATLAB Function  TreatAsAtomicUnit=on
  MATLAB Function4 : MATLAB Function  TreatAsAtomicUnit=on
  Product : Product
  Scope : Scope  Commented=on
      settings: ActiveDisplayYMinimum=-22308.19804574037  ActiveDisplayYMaximum=11892.944291168513  DataLoggingVariableName=ScopeData28
  Scope2 : Scope  Commented=on
      settings: ActiveDisplayYMinimum=-120826.17462841458  ActiveDisplayYMaximum=34452.37997376953  DataLoggingVariableName=ScopeData46
  Sum : Sum  Inputs=|++
  Sum1 : Sum  Inputs=|++
  ox_axial_f : Outport
  ox_slosh_x : Outport  Port=2
  ox_slosh_mass_x : Outport  Port=3
  ox_slosh_torque_x : Outport  Port=4
  wires:
  ox_axial_accel/1 -> MATLAB Function/1(ox_axial_accel)
  ox_axial_pendulum_l/1 -> MATLAB Function/2(ox_axial_pendulum_l), Product/2, MATLAB Function4/3(ox_axial_pendulum_l), MATLAB Function3/3(ox_axial_pendulum_l)
  Integrator/1 -> MATLAB Function2/1(ox_axial_phi_dot), Integrator1/1
  MATLAB Function2/1(velo_term) -> Sum/2
  ox_axial_natural_freq/1 -> MATLAB Function2/2(ox_axial_natural_freq), MATLAB Function1/2(ox_axial_natural_freq)
  ox_axial_damping/1 -> MATLAB Function2/3(ox_axial_damping)
  Sum/1 -> Sum1/1
  MATLAB Function1/1(ang_term) -> Scope2/1, Sum1/2
  MATLAB Function/1(accel_term) -> Sum/1
  Sum1/1 -> Integrator/1, MATLAB Function4/4(slosh_angular_accel), MATLAB Function3/1(ox_axial_phi_ddot), Scope/1
  ox_axial_slosh_mass/1 -> MATLAB Function3/2(ox_axial_slosh_mass), ox_slosh_mass_x/1, MATLAB Function4/2(ox_axial_slosh_mass)
  MATLAB Function3/1(ox_axial_f) -> ox_axial_f/1
  IC/1 -> Product/1, MATLAB Function1/1(ox_axial_phi)
  Integrator1/1 -> IC/1
  Product/1 -> ox_slosh_x/1
  x_omega_dot/1 -> MATLAB Function4/1(x_omega_dot)
  MATLAB Function4/1(x_slosh_torque) -> ox_slosh_torque_x/1

== system hopper_6dof_NED_fault_injection/Slosh/Oxidizer Pitch Force ==
  ox_pitch_accel : Inport
  ox_lateral_damping : Inport  Port=2
  ox_lateral_pendulum_l : Inport  Port=3
  ox_lateral_natural_freq : Inport  Port=4
  ox_lateral_slosh_mass : Inport  Port=5
  z_omega_dot : Inport  Port=6
  IC : InitialCondition  Value=0
  Integrator : Integrator
  Integrator1 : Integrator
  MATLAB Function : MATLAB Function  TreatAsAtomicUnit=on
  MATLAB Function1 : MATLAB Function  TreatAsAtomicUnit=on
  MATLAB Function2 : MATLAB Function  TreatAsAtomicUnit=on
  MATLAB Function3 : MATLAB Function  TreatAsAtomicUnit=on
  MATLAB Function4 : MATLAB Function  TreatAsAtomicUnit=on
  Product : Product
  Sum : Sum  Inputs=|++
  Sum1 : Sum  Inputs=|++
  ox_pitch_f : Outport
  ox_slosh_z : Outport  Port=2
  ox_slosh_mass_z : Outport  Port=3
  ox_slosh_torque_z : Outport  Port=4
  wires:
  ox_pitch_accel/1 -> MATLAB Function/1(ox_pitch_accel)
  ox_lateral_pendulum_l/1 -> MATLAB Function/2(ox_lateral_pendulum_l), Product/2, MATLAB Function4/3(ox_lateral_pendulum_l), MATLAB Function3/3(ox_lateral_pendulum_l)
  Integrator/1 -> MATLAB Function2/1(ox_pitch_phi_dot), Integrator1/1
  MATLAB Function2/1(velo_term) -> Sum/2
  ox_lateral_natural_freq/1 -> MATLAB Function1/2(ox_lateral_natural_freq), MATLAB Function2/2(ox_lateral_natural_freq)
  ox_lateral_damping/1 -> MATLAB Function2/3(ox_lateral_damping)
  Integrator1/1 -> IC/1
  Sum/1 -> Sum1/1
  MATLAB Function1/1(ang_term) -> Sum1/2
  MATLAB Function/1(accel_term) -> Sum/1
  Sum1/1 -> Integrator/1, MATLAB Function4/4(slosh_angular_accel), MATLAB Function3/1(ox_pitch_phi_ddot)
  ox_lateral_slosh_mass/1 -> ox_slosh_mass_z/1, MATLAB Function4/2(ox_lateral_slosh_mass), MATLAB Function3/2(ox_lateral_slosh_mass)
  MATLAB Function3/1(ox_pitch_f) -> ox_pitch_f/1
  IC/1 -> Product/1, MATLAB Function1/1(ox_pitch_phi)
  Product/1 -> ox_slosh_z/1
  z_omega_dot/1 -> MATLAB Function4/1(z_omega_dot)
  MATLAB Function4/1(z_slosh_torque) -> ox_slosh_torque_z/1

== system hopper_6dof_NED_fault_injection/Slosh/Oxidizer Yaw Force ==
  ox_yaw_accel : Inport
  ox_lateral_damping : Inport  Port=2
  ox_lateral_pendulum_l : Inport  Port=3
  ox_lateral_natural_freq : Inport  Port=4
  ox_lateral_slosh_mass : Inport  Port=5
  y_omega_dot : Inport  Port=6
  IC : InitialCondition  Value=0
  Integrator : Integrator
  Integrator1 : Integrator
  MATLAB Function : MATLAB Function  TreatAsAtomicUnit=on
  MATLAB Function1 : MATLAB Function  TreatAsAtomicUnit=on
  MATLAB Function2 : MATLAB Function  TreatAsAtomicUnit=on
  MATLAB Function3 : MATLAB Function  TreatAsAtomicUnit=on
  MATLAB Function4 : MATLAB Function  TreatAsAtomicUnit=on
  Product : Product
  Sum : Sum  Inputs=|++
  Sum1 : Sum  Inputs=|++
  ox_yaw_f : Outport
  ox_slosh_y : Outport  Port=2
  ox_slosh_mass_y : Outport  Port=3
  ox_slosh_torque_y : Outport  Port=4
  wires:
  ox_yaw_accel/1 -> MATLAB Function/1(ox_yaw_accel)
  ox_lateral_pendulum_l/1 -> MATLAB Function/2(ox_lateral_pendulum_l), Product/2, MATLAB Function4/3(ox_lateral_pendulum_l), MATLAB Function3/3(ox_lateral_pendulum_l)
  Integrator/1 -> MATLAB Function2/1(ox_yaw_phi_dot), Integrator1/1
  MATLAB Function2/1(velo_term) -> Sum/2
  ox_lateral_natural_freq/1 -> MATLAB Function2/2(ox_lateral_natural_freq), MATLAB Function1/2(ox_lateral_natural_freq)
  ox_lateral_damping/1 -> MATLAB Function2/3(ox_lateral_damping)
  Integrator1/1 -> IC/1
  Sum/1 -> Sum1/1
  MATLAB Function1/1(ang_term) -> Sum1/2
  MATLAB Function/1(accel_term) -> Sum/1
  Sum1/1 -> Integrator/1, MATLAB Function4/4(slosh_angular_accel), MATLAB Function3/1(ox_yaw_phi_ddot)
  ox_lateral_slosh_mass/1 -> ox_slosh_mass_y/1, MATLAB Function4/2(ox_lateral_slosh_mass), MATLAB Function3/2(ox_lateral_slosh_mass)
  MATLAB Function3/1(ox_yaw_f) -> ox_yaw_f/1
  IC/1 -> MATLAB Function1/1(ox_yaw_phi), Product/1
  Product/1 -> ox_slosh_y/1
  MATLAB Function4/1(y_slosh_torque) -> ox_slosh_torque_y/1
  y_omega_dot/1 -> MATLAB Function4/1(y_omega_dot)

== system hopper_6dof_NED_fault_injection/Slosh/Subsystem ==
  a_cg : Inport
  omega : Inport  Port=2
  omega_dot : Inport  Port=3
  r_ox_tank : Inport  Port=4
  Angular Acceleration : matrix_library/Cross Product
  Centrifugal Acceleration : matrix_library/Cross Product
  Pre-Centrifugal : matrix_library/Cross Product
  Sum : Sum  Inputs=|++
  Sum1 : Sum  Inputs=|++
  ox_a_eff : Outport
  wires:
  r_ox_tank/1 -> Pre-Centrifugal/2, Angular Acceleration/2
  omega_dot/1 -> Angular Acceleration/1
  omega/1 -> Centrifugal Acceleration/1, Pre-Centrifugal/1
  Pre-Centrifugal/1 -> Centrifugal Acceleration/2
  Centrifugal Acceleration/1 -> Sum/1
  Angular Acceleration/1 -> Sum/2
  Sum/1 -> Sum1/1
  a_cg/1 -> Sum1/2
  Sum1/1 -> ox_a_eff/1

== system hopper_6dof_NED_fault_injection/Slosh/Subsystem1 ==
  a_cg : Inport
  omega : Inport  Port=2
  omega_dot : Inport  Port=3
  r_fu_tank : Inport  Port=4
  Angular Acceleration : matrix_library/Cross Product
  Centrifugal Acceleration : matrix_library/Cross Product
  Pre-Centrifugal : matrix_library/Cross Product
  Sum : Sum  Inputs=|++
  Sum1 : Sum  Inputs=|++
  fu_a_eff : Outport
  wires:
  r_fu_tank/1 -> Pre-Centrifugal/2, Angular Acceleration/2
  omega_dot/1 -> Angular Acceleration/1
  omega/1 -> Centrifugal Acceleration/1, Pre-Centrifugal/1
  Pre-Centrifugal/1 -> Centrifugal Acceleration/2
  Centrifugal Acceleration/1 -> Sum/1
  Angular Acceleration/1 -> Sum/2
  Sum/1 -> Sum1/1
  a_cg/1 -> Sum1/2
  Sum1/1 -> fu_a_eff/1

== system hopper_6dof_NED_fault_injection/Subsystem2/If Action Subsystem ==
  Thrust : Inport
  Action Port : ActionPort  ActionPortLabel=if(u1 > 0 & u2 > 0)
  Out1 : Outport
  wires:
  Thrust/1 -> Out1/1

== system hopper_6dof_NED_fault_injection/Subsystem2/If Action Subsystem1 ==
  Thrust : Inport
  Action Port : ActionPort  ActionPortLabel=else
  Gain : Gain  Gain=0
  Out1 : Outport
  wires:
  Thrust/1 -> Gain/1
  Gain/1 -> Out1/1

== system hopper_6dof_NED_fault_injection/Subsystem3/If Action Subsystem ==
  In1 : Inport
  Action Port : ActionPort  ActionPortLabel=|
      | if(u1 > -1e-3 & u2 > 0
      | )
  Delay : Delay  Commented=through
  Stop Simulation : Stop
  wires:
  In1/1 -> Delay/1
  Delay/1 -> Stop Simulation/1

== system hopper_6dof_NED_fault_injection/Subsystem4/If Action Subsystem ==
  Thrust : Inport
  Action Port : ActionPort  ActionPortLabel=else
  Out1 : Outport
  wires:
  Thrust/1 -> Out1/1

== system hopper_6dof_NED_fault_injection/Subsystem4/If Action Subsystem1 ==
  Thrust : Inport
  Action Port : ActionPort  ActionPortLabel=if(u1 > -0.1 & u2 > 0)
  Clock : Clock
  Compare To Constant : simulink/Logic and Bit Operations/Compare To Constant  relop=<=  const=5  OutDataTypeStr=boolean
  Product : Product
  Out1 : Outport
  wires:
  Thrust/1 -> Product/1
  Product/1 -> Out1/1
  Clock/1 -> Compare To Constant/1
  Compare To Constant/1 -> Product/2

== system hopper_6dof_NED_fault_injection/Wind Forces/If Action Subsystem ==
  In1 : Inport
  Action Port : ActionPort  ActionPortLabel=if(u1 == 1)
  Constant : Constant  Value=IN.wind.uwind
  Constant1 : Constant  Value=IN.wind.vwind
  Mux : Mux  Inputs=2
  Terminator : Terminator
  Out1 : Outport
  wires:
  In1/1 -> Terminator/1
  Constant/1 -> Mux/1
  Constant1/1 -> Mux/2
  Mux/1 -> Out1/1

== system hopper_6dof_NED_fault_injection/Wind Forces/If Action Subsystem1 ==
  In1 : Inport
  Action Port : ActionPort  ActionPortLabel=elseif(u1 == 2)
  Constant : Constant  Value=IN.wind.uwind
  Constant1 : Constant  Value=IN.wind.vwind
  Constant3 : Constant  Value=[10;20]
  Mux : Mux  Inputs=2
  Terminator : Terminator
  Out2 : Outport
  wires:
  In1/1 -> Terminator/1
  Mux/1 -> Out2/1
  Constant/1 -> Mux/1
  Constant1/1 -> Mux/2

== system hopper_6dof_NED_fault_injection/Wind Forces/If Action Subsystem2 ==
  In1 : Inport
  Action Port : ActionPort  ActionPortLabel=else
  Display : Display
  Display1 : Display
  Latitude : Constant  Value=33.78
  Longitude : Constant  Value=84.40
  Month : Constant  Value=4
  Mux : Mux  Inputs=2
  Pressure (mb) : Constant  Value=1000
  Terminator : Terminator
  n-D Lookup Table : Lookup_n-D  NumberOfTableDimensions=4  BreakpointsForDimension1=1:12  BreakpointsForDimension2=pressureLevels  BreakpointsForDimension3=[32.5 35]  BreakpointsForDimension4=[82.5 85]  Table=uwndTable  ExtrapMethod=Clip  InternalRulePriority=Speed  RndMeth=Simplest
      settings: InputPortMap=u0,u1,u2,u3
  n-D Lookup Table1 : Lookup_n-D  NumberOfTableDimensions=4  BreakpointsForDimension1=1:12  BreakpointsForDimension2=pressureLevels  BreakpointsForDimension3=[32.5 35]  BreakpointsForDimension4=[82.5 85]  Table=vwndTable  InternalRulePriority=Speed  RndMeth=Simplest
      settings: InputPortMap=u0,u1,u2,u3
  Out1 : Outport
  wires:
  Month/1 -> n-D Lookup Table1/1, n-D Lookup Table/1
  Pressure (mb)/1 -> n-D Lookup Table1/2, n-D Lookup Table/2
  Latitude/1 -> n-D Lookup Table1/3, n-D Lookup Table/3
  In1/1 -> Terminator/1
  Longitude/1 -> n-D Lookup Table1/4, n-D Lookup Table/4
  n-D Lookup Table/1 -> Display/1, Mux/1
  n-D Lookup Table1/1 -> Display1/1, Mux/2
  Mux/1 -> Out1/1

== system hopper_6dof_NED_fault_injection/Fluid Network2/COPV/COPV Leakage ==
  Leak Rate : fl_lib/Gas/Elements/Flow Resistance (G)  delta_p_nominal=0.001 MPa  mdot_nominal=0.0000000001 kg/s  rho_nominal=0 kg/m^3  area=0.01 m^2  laminar_fraction=1e-3
      settings: InternalSimscapePortConfiguration="{\"Bottom\":[],\"Left\":[{\"id\":\"A\",\"label\":\"A\",\"type\":\"foundation.gas.gas\"}],\"Right\":[{\"id\":\"B\",\"label\":\"B\",\"type\":\"foundation.gas.gas\"}],\"Top\":[]}"
  Mass & Energy Flow Rate Sensor (G)2 : fl_lib/Gas/Sensors/Flow Rate Sensor (G)  mass_flow_measure=true  volumetric_flow_measure=false  volumetric_flow_conditions=foundation.enum.volumetric_flow_conditions.actual  p_std=0.101325 MPa  T_std=20 degC  energy_flow_measure=true
      settings: InternalSimscapePortConfiguration="{\"Bottom\":[{\"id\":\"PHI\",\"label\":\"φ\",\"type\":\"output\"}],\"Left\":[{\"id\":\"A\",\"label\":\"A\",\"type\":\"foundation.gas.gas\"}],\"Right\":[{\"id\":\"B\",\"label\":\"B\",\"type\":\"foundation.gas.gas\"},{\"id\":\"M\",\"label\":\"M\",\"type\":\"output\"}],\"Top\":[]}"
  PS-Simulink Converter7 : nesl_utility/PS-Simulink Converter  PhysicalDomain=network_engine_domain  SubClassName=ps_output  LeftPortType=input  RightPortType=output  PseudoPeriodic=off  Frequencies=[]  VectorFormat=inherit  Unit=inherit  AffineConversion=off
  Pressurant Mass Leak Rate : Scope  Commented=on
      settings: ActiveDisplayYMinimum=-1  ActiveDisplayYMaximum=1
  Reservoir (G) : fl_lib/Gas/Elements/Reservoir (G)  pressure_spec=foundation.enum.pressure_spec.atmospheric  reservoir_pressure=0.101325 MPa  reservoir_temperature=293.15 K  area_A=0.01 m^2
  Conn1 : PMIOPort  Side=Right
  wires:
  PS-Simulink Converter7/1 -> Pressurant Mass Leak Rate/1
  connections:
  Conn1/RConn1 -- Leak Rate/RConn1
  Leak Rate/LConn1 -- Mass & Energy Flow Rate Sensor (G)2/LConn1
  Mass & Energy Flow Rate Sensor (G)2/RConn1 -- Reservoir (G)/LConn1
  Mass & Energy Flow Rate Sensor (G)2/RConn2 -- PS-Simulink Converter7/LConn1
